simulink model "Exp1"  (R2025b)
settings: Solver=VariableStepAuto  StartTime=0.0  StopTime=10.0  RelTol=1e-3
libraries: simulink_extras x5
settings Model: Creator=SUBHASH  LastModifiedBy=SUBHASH

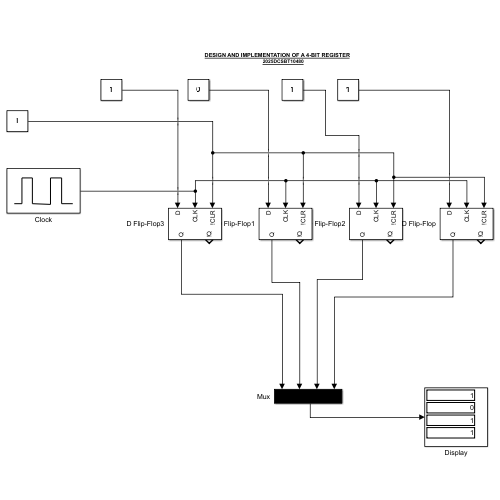
[thumbnail: Simulink's stored preview of the top-level diagram]
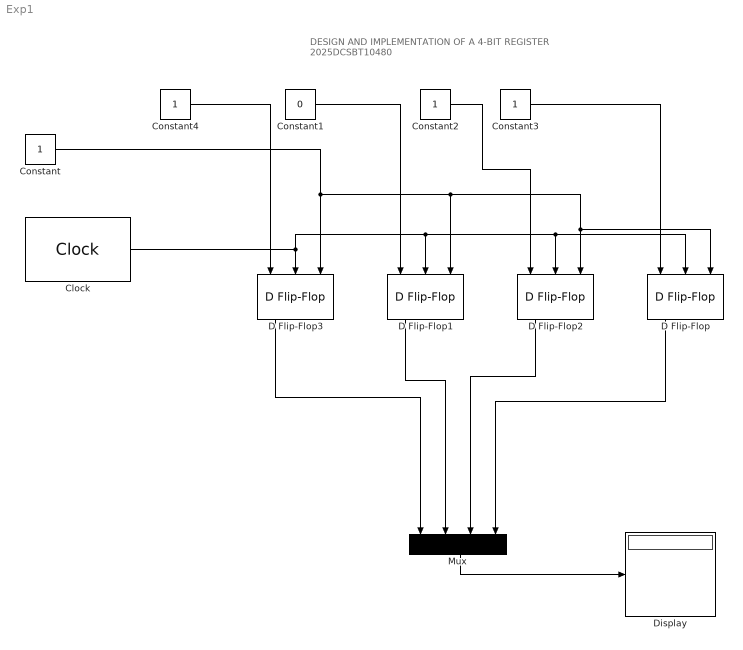
== system Exp1 ==
  note: DESIGN AND IMPLEMENTATION OF A 4-BIT REGISTER
      | 2025DCSBT10480
  Clock : simulink_extras/Flip Flops/Clock  period=2
  Constant{,2..4} (4 alike) : Constant  OutDataTypeStr=boolean
  Constant1 : Constant  Value=0  OutDataTypeStr=boolean
  D Flip-Flop{,1..3} (4 alike) : simulink_extras/Flip Flops/D Flip-Flop
  Display : Display
  Mux : Mux
  wires:
  Constant/1 -> D Flip-Flop3/3, D Flip-Flop1/3, D Flip-Flop/3, D Flip-Flop2/3
  Clock/1 -> D Flip-Flop1/2, D Flip-Flop/2, D Flip-Flop2/2, D Flip-Flop3/2
  Constant4/1 -> D Flip-Flop3/1
  Constant1/1 -> D Flip-Flop1/1
  Constant2/1 -> D Flip-Flop2/1
  Constant3/1 -> D Flip-Flop/1
  D Flip-Flop1/1 -> Mux/2
  D Flip-Flop2/1 -> Mux/3
  D Flip-Flop/1 -> Mux/4
  D Flip-Flop3/1 -> Mux/1
  Mux/1 -> Display/1
